simulink model "Complete_SAD_model"  (R2025b)
settings: Solver=ode4  StartTime=0.0  StopTime=10  FixedStep=0.01  RelTol=1e-3
values from neighbouring files (symbols this model uses):
  A = eye(3)    [Initial_condition.m]
  a_pink = exp(-2*pi*fc_pink*Ts_m*k_pink)    [Initial_condition.m]
  acc = deg2rad(0.5*randn)    [Initial_condition.m]
  Ap = eye(3)    [Initial_condition.m]
  D = 500*10^-12    (= 5e-10)    [Initial_condition.m]
  delay = 1    [Initial_condition.m]
  inv_Ir = inv(Ir)    [Initial_condition.m]
  Ir = diag([Irx,Iry,Irz])    [Initial_condition.m]
  J_B = diag([Ix,Iy,Iz])    [Initial_condition.m]
  m = [0.01; 0.01; 0.01]    [Initial_condition.m]
  m_max = [0.65; 0.65; 0.5]    [Initial_condition.m]
  Mr_max = [0.01; 0.01; 0.01]    [Initial_condition.m]
  mu_earth = 398600.433    [Initial_condition.m]
  mu_sun = 132712440017.987    (= 132712440018)    [Initial_condition.m]
  non_ort = deg2rad(-1+2*rand)    [Initial_condition.m]
  omega0 = [wx;wy;wz]    [Initial_condition.m]
  rES0_ECI = [0 AU 0]    [Initial_condition.m]
  seed = 0    [Initial_condition.m]
  sigma = (2*pi/60)/3    (= 0.0349065850399)    [Initial_condition.m]
  Ts_m = 1/f_m    (= 0.1)    [Initial_condition.m]
  Ts_ss = 1/f_ss    (= 0.1)    [Initial_condition.m]
  vES0_ECI = [(-sqrt(mu_sun/norm(rES0_ECI))) 0 0 ]    [Initial_condition.m]
  w_max = [250; 250; 250]    [Initial_condition.m]
undefined symbols (not defined in the file or in its folder): dspblkCoreblockFVToolHelper, gcbh, K, r0_ECI, v0_ECI
libraries: matrix_library x15, dspmathops x3, dspfdesign x3, vrlib x2
(part 2 of 3)

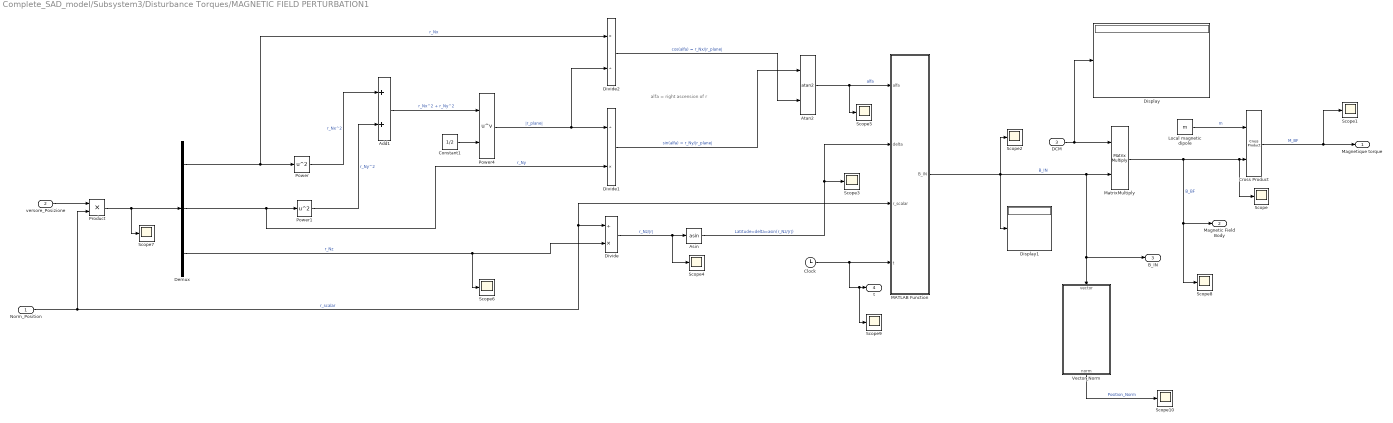
== system Complete_SAD_model/Subsystem3/Disturbance Torques/MAGNETIC FIELD PERTURBATION1 ==
  note: alfa = right ascension of r
  Norm_Position : Inport
  versore_Posizione : Inport  Port=2
  DCM : Inport  Port=3
  Add1 : Sum
  Asin : Trigonometry  Operator=asin
  Atan2 : Trigonometry  Operator=atan2
  Clock : Clock
  Constant1 : Constant  Value=1/2
  Cross Product : matrix_library/Cross Product
  Demux : Demux  Outputs=3
  Display : Display
  Display1 : Display
  Divide : Product  Inputs=/*
  Divide1 : Product  Inputs=/*
  Divide2 : Product  Inputs=*/
  Local magnetic dipole : Constant  Value=m
  MATLAB Function : MATLAB Function  TreatAsAtomicUnit=on
  MatrixMultiply : Product  Multiplication=Matrix(*)
  Power : Math  Operator=square
  Power1 : Math  Operator=square
  Power4 : Math  Operator=pow
  Product : Product
  Scope{,1..10} (11 alike) : Scope
      Scope settings: ActiveDisplayYMinimum=-1.9912639141630993E-5  ActiveDisplayYMaximum=7.6680141837987377E-5
      Scope1 settings: ActiveDisplayYMinimum=-1  ActiveDisplayYMaximum=1  DataLoggingVariableName=ScopeData18
      Scope10 settings: DataLoggingVariableName=ScopeData41
      Scope2 settings: ActiveDisplayYMinimum=-7.927665187698622E-5  ActiveDisplayYMaximum=7.2341602666760142E-5  DataLoggingVariableName=ScopeData7
      Scope3 settings: ActiveDisplayYMinimum=1.0779442647435169  ActiveDisplayYMaximum=1.615926279910795  DataLoggingVariableName=ScopeData6
      Scope4 settings: DataLoggingVariableName=ScopeData15
      Scope5 settings: ActiveDisplayYMinimum=-3.9269905541818266  ActiveDisplayYMaximum=3.9269896027954103  DataLoggingVariableName=ScopeData19
      Scope6 settings: ActiveDisplayYMinimum=-7471.456381733512  ActiveDisplayYMaximum=7471.4563817894887  DataLoggingVariableName=ScopeData20
      Scope7 settings: ActiveDisplayYMinimum=-7505.9997864225315  ActiveDisplayYMaximum=7493.99997626917  DataLoggingVariableName=ScopeData21
      Scope8 settings: ActiveDisplayYMinimum=-6.8946774907106514E-5  ActiveDisplayYMaximum=6.710524246748423E-5  DataLoggingVariableName=ScopeData23
      Scope9 settings: DataLoggingVariableName=ScopeData52
  Vector_Norm : Subsystem
  Magnetique torque : Outport
  Magnetic Field Body : Outport  Port=2
  B_IN : Outport  Port=3
  t : Outport  Port=4
  wires:
  Cross Product/1 -> Scope1/1, Magnetique torque/1  "M_BF"
  MatrixMultiply/1 -> Scope8/1, Magnetic Field Body/1, Scope/1, Cross Product/2  "B_BF"
  Local magnetic dipole/1 -> Cross Product/1  "m"
  Asin/1 -> Scope3/1, MATLAB Function/2(delta)  "Latitude=delta=asin(r_Nz/|r|)"
  Atan2/1 -> Scope5/1, MATLAB Function/1(alfa)  "alfa"
  Demux/2 -> Power1/1, Divide1/2  "r_Ny"
  Demux/3 -> Scope6/1, Divide/2  "r_Nz"
  MATLAB Function/1(B_IN) -> Scope2/1, Vector_Norm/1(vector), B_IN/1, MatrixMultiply/2, Display1/1  "B_IN"
  Divide1/1 -> Atan2/1  "sin(alfa) = r_Ny/|r_plane|"
  DCM/1 -> MatrixMultiply/1, Display/1
  Add1/1 -> Power4/1  "r_Nx^2 + r_Ny^2"
  Power/1 -> Add1/1  "r_Nx^2"
  Constant1/1 -> Power4/2
  Demux/1 -> Power/1, Divide2/1  "r_Nx"
  Power1/1 -> Add1/2  "r_Ny^2"
  Divide2/1 -> Atan2/2  "cos(alfa) = r_Nx/|r_plane|"
  Divide/1 -> Scope4/1, Asin/1  "r_Nz/|r|"
  Power4/1 -> Divide1/1, Divide2/2  "|r_plane|"
  Clock/1 -> MATLAB Function/4(t), Scope9/1, t/1
  Norm_Position/1 -> Product/2, MATLAB Function/3(r_scalar), Divide/1  "r_scalar"
  versore_Posizione/1 -> Product/1
  Product/1 -> Scope7/1, Demux/1
  Vector_Norm/1(norm) -> Scope10/1  "Position_Norm"

== system Complete_SAD_model/Subsystem3/Orbita Propagation1/ Earth - Sun Two - Body ==
  Constant : Constant  Value=3
  Constant1 : Constant  Value=-mu_sun
  Integrator : Integrator  InitialCondition=vES0_ECI
  Integrator1 : Integrator  InitialCondition=rES0_ECI
  Math Function : Math  Operator=pow
  Product : Product  Inputs=**/
  To Workspace : ToWorkspace  VariableName=v_ECI_sun  SampleTime=-1
  To Workspace1 : ToWorkspace  VariableName=r_ES_ECI  SampleTime=-1
  Vector_Norm : Subsystem
  Position Earth - Sun : Outport
  wires:
  Product/1 -> Integrator/1  "Acceleration"
  Math Function/1 -> Product/3
  Constant1/1 -> Product/2
  Vector_Norm/1(norm) -> Math Function/1  "Position_Norm"
  Integrator/1 -> Integrator1/1, To Workspace/1  "Velocity"
  Integrator1/1 -> Product/1, Vector_Norm/1(vector), To Workspace1/1, Position Earth - Sun/1  "r_ES_ECI"
  Constant/1 -> Math Function/2

== system Complete_SAD_model/Subsystem3/Orbita Propagation1/Spacecraft - Earth Two - Body ==
  Constant : Constant  Value=3
  Constant1 : Constant  Value=-mu_earth
  Cross Product : matrix_library/Cross Product
  Integrator : Integrator  InitialCondition=v0_ECI
  Integrator1 : Integrator  InitialCondition=r0_ECI
  Math Function : Math  Operator=pow
  Product : Product  Inputs=**/
  Product1 : Product  Inputs=*/
  To Workspace : ToWorkspace  VariableName=v_ECI  SampleTime=-1
  To Workspace2 : ToWorkspace  VariableName=r_ECI  SampleTime=-1
  Vector_Norm : Subsystem
  Position Spacecraft .- Earth : Outport
  "Norm of Position Spacecraft - Earth " : Outport  Port=2
  h vector : Outport  Port=3
  Versore Posizione : Outport  Port=4
  wires:
  Product1/1 -> Versore Posizione/1
  Product/1 -> Integrator/1  "Acceleration"
  Integrator1/1 -> Cross Product/1, Product/1, Vector_Norm/1(vector), Product1/1, To Workspace2/1, Position Spacecraft .- Earth/1  "Position"
  Integrator/1 -> Integrator1/1, To Workspace/1, Cross Product/2  "Velocity"
  Vector_Norm/1(norm) -> Math Function/1, Product1/2, "Norm of Position Spacecraft - Earth "/1  "Position_Norm"
  Constant/1 -> Math Function/2
  Math Function/1 -> Product/3
  Constant1/1 -> Product/2
  Cross Product/1 -> h vector/1

== system Complete_SAD_model/Subsystem/Determination Algorithm/ALGEBRAIC METHOD for ATTITUDE DETERMINATION 1/Subsystem ==
  p x q : Inport
  Sqrt : Sqrt
  Square : Math  Operator=square
  Sum of Elements : Sum  Inputs=+
  |p x q| : Outport
  wires:
  p x q/1 -> Square/1
  Sqrt/1 -> |p x q|/1
  Square/1 -> Sum of Elements/1
  Sum of Elements/1 -> Sqrt/1

== system Complete_SAD_model/Subsystem/Determination Algorithm/ALGEBRAIC METHOD for ATTITUDE DETERMINATION 1/Subsystem1 ==
  a x b : Inport
  Sqrt1 : Sqrt
  Square1 : Math  Operator=square
  Sum of Elements1 : Sum  Inputs=+
  |a x b| : Outport
  wires:
  a x b/1 -> Square1/1
  Sum of Elements1/1 -> Sqrt1/1
  Square1/1 -> Sum of Elements1/1
  Sqrt1/1 -> |a x b|/1

== system Complete_SAD_model/Subsystem/Subsystem2/MAGNETOMETER/Brown noise ==
  Gain1 : Gain  Gain=D/sqrt(2*Ts_m)
  Gain2 : Gain  Gain=D/sqrt(2*Ts_m)
  Gain3 : Gain  Gain=D/sqrt(2*Ts_m)
  Lowpass Filter 6dB/oct : dspfdesign/Lowpass Filter  FilterType=FIR  DesignForMinimumOrder=on  FilterOrder=50  PassbandFrequency=0.3628  StopbandFrequency=0.5442  PassbandRipple=0.1  StopbandAttenuation=80  SampleRateMode=Use normalized frequency (0 to 1)  SampleRate=44100  SimulateUsing=Interpreted execution  roundingMode=Floor  coeffsDataTypeStr=fixdt(1,16)
  Lowpass Filter 6dB/oct1 : dspfdesign/Lowpass Filter  FilterType=IIR  DesignForMinimumOrder=off  FilterOrder=1  PassbandFrequency=0.1  StopbandFrequency=0.5442  PassbandRipple=0.1  StopbandAttenuation=80  SampleRate=44100  SimulateUsing=Interpreted execution  roundingMode=Floor  coeffsDataTypeStr=fixdt(1,16)
  Lowpass Filter 6dB/oct2 : dspfdesign/Lowpass Filter  FilterType=IIR  DesignForMinimumOrder=off  FilterOrder=1  PassbandFrequency=0.1  StopbandFrequency=0.5442  PassbandRipple=0.1  StopbandAttenuation=80  SampleRate=44100  SimulateUsing=Interpreted execution  roundingMode=Floor  coeffsDataTypeStr=fixdt(1,16)
  Mux4 : Mux  Inputs=3
  Random Number2 : RandomNumber  Seed=seed+3  SampleTime=Ts_m
  Random Number4 : RandomNumber  Seed=seed+4  SampleTime=Ts_m
  Random Number5 : RandomNumber  Seed=seed+5  SampleTime=Ts_m
  Scope1 : Scope
      settings: ActiveDisplayYMinimum=-1  ActiveDisplayYMaximum=1  DataLoggingVariableName=ScopeData13
  Brown noise : Outport
  wires:
  Lowpass Filter 6dB/oct/1 -> Mux4/3
  Random Number5/1 -> Gain2/1
  Gain2/1 -> Lowpass Filter 6dB/oct/1
  Lowpass Filter 6dB/oct1/1 -> Mux4/2
  Gain3/1 -> Lowpass Filter 6dB/oct2/1
  Random Number2/1 -> Gain3/1
  Gain1/1 -> Lowpass Filter 6dB/oct1/1
  Random Number4/1 -> Gain1/1
  Lowpass Filter 6dB/oct2/1 -> Mux4/1
  Mux4/1 -> Scope1/1, Brown noise/1  "Brown noise"

== system Complete_SAD_model/Subsystem/Subsystem2/MAGNETOMETER/Misalignement ==
  Constant : Constant  Value=non_ort
  Constant1 : Constant  Value=0
  Constant2 : Constant  Value=-non_ort
  Constant3 : Constant  Value=eye(3)
  Minus : Sum  Inputs=+-
  Mux : Mux  Inputs=3
  Mux1 : Mux  Inputs=3
  Mux2 : Mux  Inputs=3
  Vector Concatenate : Concatenate  NumInputs=3  Mode=Multidimensional array  ConcatenateDimension=2
  misalignement_error : Outport
  wires:
  Mux1/1 -> Vector Concatenate/2
  Mux2/1 -> Vector Concatenate/3
  Mux/1 -> Vector Concatenate/1
  Minus/1 -> misalignement_error/1  "misalignement_error"
  Constant3/1 -> Minus/1
  Constant1/1 -> Mux/1, Mux1/2, Mux2/3
  Constant2/1 -> Mux1/1, Mux/3, Mux2/2
  Vector Concatenate/1 -> Minus/2
  Constant/1 -> Mux/2, Mux1/3, Mux2/1

== system Complete_SAD_model/Subsystem/Subsystem2/MAGNETOMETER/Pink noise ==
  Discrete Filter : DiscreteFilter  LoadFcn=dspblkCoreblockFVToolHelper(gcbh,'load');  Numerator=[1-a_pink]  Denominator=[1 -a_pink]
      settings: CopyFcn=dspblkCoreblockFVToolHelper(gcbh,'copy');  DeleteFcn=dspblkCoreblockFVToolHelper(gcbh,'close');  ModelCloseFcn=dspblkCoreblockFVToolHelper(gcbh,'close');  PreSaveFcn=dspblkCoreblockFVToolHelper(gcbh,'presave');  PostSaveFcn=dspblkCoreblockFVToolHelper(gcbh,'postsave');  CloseFcn=dspblkCoreblockFVToolHelper(gcbh,'close');
  Discrete Filter1 : DiscreteFilter  LoadFcn=dspblkCoreblockFVToolHelper(gcbh,'load');  Numerator=[1-a_pink]  Denominator=[1 -a_pink]
      settings: CopyFcn=dspblkCoreblockFVToolHelper(gcbh,'copy');  DeleteFcn=dspblkCoreblockFVToolHelper(gcbh,'close');  ModelCloseFcn=dspblkCoreblockFVToolHelper(gcbh,'close');  PreSaveFcn=dspblkCoreblockFVToolHelper(gcbh,'presave');  PostSaveFcn=dspblkCoreblockFVToolHelper(gcbh,'postsave');  CloseFcn=dspblkCoreblockFVToolHelper(gcbh,'close');
  Discrete Filter2 : DiscreteFilter  Numerator=[1-a_pink]  Denominator=[1 -a_pink]
  Gain4 : Gain  Gain=D/sqrt(2*Ts_m)
  Gain5 : Gain  Gain=D/sqrt(2*Ts_m)
  Gain6 : Gain  Gain=D/sqrt(2*Ts_m)
  Mux5 : Mux  Inputs=3
  Random Number6 : RandomNumber  Seed=seed + 6  SampleTime=Ts_m
  Random Number7 : RandomNumber  Seed=seed+7  SampleTime=Ts_m
  Random Number8 : RandomNumber  Seed=seed+8  SampleTime=Ts_m
  Scope4 : Scope
      settings: ActiveDisplayYMinimum=-1  ActiveDisplayYMaximum=1  DataLoggingVariableName=ScopeData16
  pink noise : Outport
  wires:
  Gain5/1 -> Discrete Filter1/1
  Random Number6/1 -> Gain6/1  "asse X"
  Random Number7/1 -> Gain5/1  "asse Y"
  Discrete Filter/1 -> Mux5/1
  Discrete Filter1/1 -> Mux5/2
  Mux5/1 -> Scope4/1, pink noise/1  "pink noise"
  Discrete Filter2/1 -> Mux5/3
  Gain4/1 -> Discrete Filter2/1
  Gain6/1 -> Discrete Filter/1
  Random Number8/1 -> Gain4/1  "asse Z"

== system Complete_SAD_model/Subsystem/Subsystem2/MAGNETOMETER/White noise ==
  Gain : Gain  Gain=D/sqrt(2*Ts_m)
  Mux3 : Mux  Inputs=3
  Random Number : RandomNumber  Seed=seed  SampleTime=Ts_m
  Random Number1 : RandomNumber  Seed=seed+1  SampleTime=Ts_m
  Random Number3 : RandomNumber  Seed=seed+2  SampleTime=Ts_m
  Scope2 : Scope
      settings: ActiveDisplayYMinimum=-1  ActiveDisplayYMaximum=1  DataLoggingVariableName=ScopeData14
  white noise : Outport
  wires:
  Random Number1/1 -> Mux3/2
  Random Number/1 -> Mux3/1
  Mux3/1 -> Gain/1
  Random Number3/1 -> Mux3/3
  Gain/1 -> Scope2/1, white noise/1  "white noise"

== system Complete_SAD_model/Subsystem3/Attitude Kinematics  with orthonormalization/A_L|N/Vector_Norm ==
  vector : Inport
  Add : Sum  Inputs=+++
  Demux : Demux  Outputs=3
  Sqrt : Sqrt
  Square : Math  Operator=square
  Square1 : Math  Operator=square
  Square2 : Math  Operator=square
  norm : Outport
  wires:
  Sqrt/1 -> norm/1  "norm"
  Demux/2 -> Square1/1  "r_y"
  Add/1 -> Sqrt/1
  Square2/1 -> Add/3  "r_z^2"
  Demux/1 -> Square/1  "r_x"
  Demux/3 -> Square2/1  "r_z"
  Square1/1 -> Add/2  "r_y^2"
  Square/1 -> Add/1  "r_x^2"
  vector/1 -> Demux/1

== system Complete_SAD_model/Subsystem3/Disturbance Torques/MAGNETIC FIELD PERTURBATION1/Vector_Norm ==
  vector : Inport
  Add : Sum  Inputs=+++
  Demux : Demux  Outputs=3
  Sqrt : Sqrt
  Square : Math  Operator=square
  Square1 : Math  Operator=square
  Square2 : Math  Operator=square
  norm : Outport
  wires:
  Sqrt/1 -> norm/1  "norm"
  Demux/2 -> Square1/1  "r_y"
  Add/1 -> Sqrt/1
  Square2/1 -> Add/3  "r_z^2"
  Demux/1 -> Square/1  "r_x"
  Demux/3 -> Square2/1  "r_z"
  Square1/1 -> Add/2  "r_y^2"
  Square/1 -> Add/1  "r_x^2"
  vector/1 -> Demux/1

== system Complete_SAD_model/Subsystem3/Orbita Propagation1/ Earth - Sun Two - Body/Vector_Norm ==
  vector : Inport
  Add : Sum  Inputs=+++
  Demux : Demux  Outputs=3
  Sqrt : Sqrt
  Square : Math  Operator=square
  Square1 : Math  Operator=square
  Square2 : Math  Operator=square
  norm : Outport
  wires:
  Sqrt/1 -> norm/1  "norm"
  Demux/2 -> Square1/1  "r_y"
  Add/1 -> Sqrt/1
  Square2/1 -> Add/3  "r_z^2"
  Demux/1 -> Square/1  "r_x"
  Demux/3 -> Square2/1  "r_z"
  Square1/1 -> Add/2  "r_y^2"
  Square/1 -> Add/1  "r_x^2"
  vector/1 -> Demux/1

== system Complete_SAD_model/Subsystem3/Orbita Propagation1/Spacecraft - Earth Two - Body/Vector_Norm ==
  vector : Inport
  Add : Sum  Inputs=+++
  Demux : Demux  Outputs=3
  Sqrt : Sqrt
  Square : Math  Operator=square
  Square1 : Math  Operator=square
  Square2 : Math  Operator=square
  norm : Outport
  wires:
  Sqrt/1 -> norm/1  "norm"
  Demux/2 -> Square1/1  "r_y"
  Add/1 -> Sqrt/1
  Square2/1 -> Add/3  "r_z^2"
  Demux/1 -> Square/1  "r_x"
  Demux/3 -> Square2/1  "r_z"
  Square1/1 -> Add/2  "r_y^2"
  Square/1 -> Add/1  "r_x^2"
  vector/1 -> Demux/1
